simulink model "inverted_pendulum_pid"  (R2022a)
settings: Solver=VariableStepAuto  StartTime=0.0  StopTime=200  RelTol=1e-3
libraries: aerolibconvert2 x2
settings Model: Creator=User
settings ModelReferenceCC: EnableRefExpFcnMdlSchedulingChecks=off
settings RTWCC: Description=Generic Real-Time Target

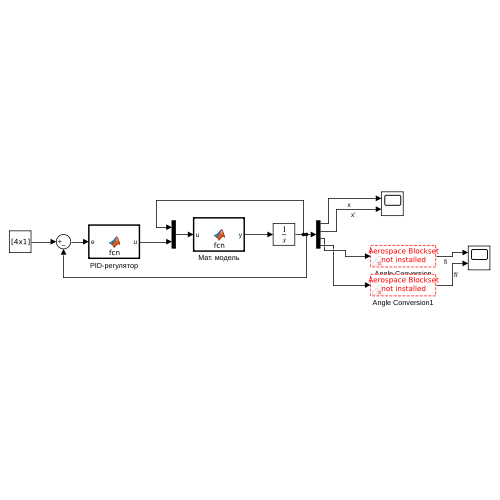
[thumbnail: Simulink's stored preview of the top-level diagram]
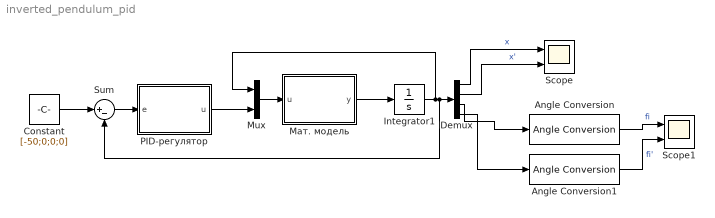
== system inverted_pendulum_pid ==
  Angle Conversion : aerolibconvert2/Angle Conversion  IU=rad  OU=deg
  Angle Conversion1 : aerolibconvert2/Angle Conversion  IU=rad  OU=deg
  Constant : Constant  Value=[-50;0;0;0]
  Demux : Demux
  Integrator1 : Integrator  InitialCondition=[0;0;0.25;0]
  Mux : Mux  Inputs=2
  PID-регулятор : MATLAB Function  TreatAsAtomicUnit=on
  Scope : Scope  NumInputPorts=2
  Scope1 : Scope  NumInputPorts=2
  Sum : Sum  Inputs=|+-
  Мат. модель : MATLAB Function  TreatAsAtomicUnit=on
  wires:
  Angle Conversion/1 -> Scope1/1  "fi"
  Мат. модель/1(y) -> Integrator1/1
  Demux/1 -> Scope/1  "x"
  Demux/2 -> Scope/2  "x'"
  Demux/3 -> Angle Conversion/1
  Demux/4 -> Angle Conversion1/1
  Angle Conversion1/1 -> Scope1/2  "fi'"
  Integrator1/1 -> Sum/2, Demux/1, Mux/1
  Mux/1 -> Мат. модель/1(u)
  Sum/1 -> PID-регулятор/1(e)
  Constant/1 -> Sum/1
  PID-регулятор/1(u) -> Mux/2

== matlab function inverted_pendulum_pid/Мат. модель ==
  data: u input; y output
function y = fcn(u)
y = zeros(4,1);

M1 = 3.3;
M2 = 2.5;
M3 = 2.3;
L = 0.3;

y(1) = u(2);
%y(2) = (0.25*u(4)*u(4)*0.3*sin(u(3))-9.81*0.3*cos(u(3))*sin(u(3)))/(3.3+cos(u(3)));
y(2) = (u(5)*M3*L*L + M2*L*sin(u(3))*(L*9.81*cos(u(3))-u(4)*M2*L*L-M2*L*cos(u(3))*0.25*u(4)))/(L*L*(M3*M1-M2*M2*cos(u(3))*cos(u(3))));
y(3) = u(4);
%y(4) = (0.25*0.3*0*cos(u(3))-0.25*0.25*0.3*0.3*u(4)*u(4)*cos(u(3))*sin(u(3))+3.3*0.25*9.81*0.3*sin(u(3))-0.01*u(4))/(3.3*0.23*0.3*0.3-0.25*0.25*0.3*0.3*cos(u(3))*cos(u(3)));
%y(2) = (u(5)-0.25*(0.3*y(4)*cos(u(3))-0.3*u(4)*u(4)*sin(u(3))))/3.3;
%y(4) = (9.81*sin(u(3))-y(2)*cos(u(3))-0.05*u(4))/0.25;
y(4) = (M2*9.81*L*sin(u(3))+M2*L*y(2)*cos(u(3))-0.25*u(4))/M3*L*L;

end

== matlab function inverted_pendulum_pid/PID-регулятор ==
  data: e input; u output
function u = fcn(e)
e(2) = - e(2);
u = 400*e(4) + 300*e(3) + 2.5*e(2);
%u(5) = 0;
end
